simulink model "brakelight_example"  (R2025b)
settings: Solver=FixedStepAuto  StartTime=0.0  StopTime=10.0  RelTol=1e-3
libraries: simulink x3
settings Model: Creator=seanmk  LastModifiedBy=seanmk
settings ConfigComp: DVMaxProcessTime=300.0  DVModelCoverageObjectives=MCDC  DVMaxTestCaseSteps=10000.0  DVTestSuiteOptimization=Auto  DVAbsoluteTolerance=1.0e-5  DVDefectChecker=on  DVDetectOutOfBounds=on  DVMaxViolationSteps=20.0  DVModelReferenceHarness=on  DVHarnessSource=Signal Editor  DVActiveTab=0.0

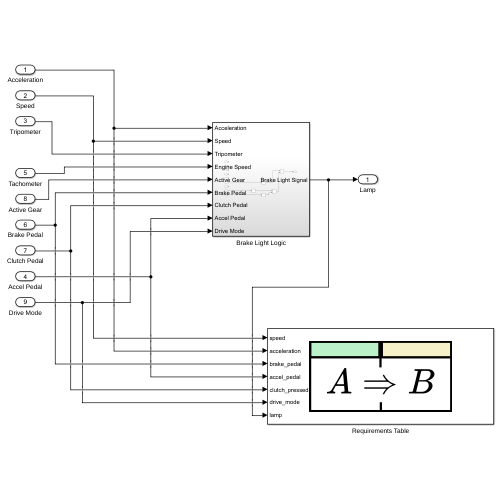
[thumbnail: Simulink's stored preview of the top-level diagram]
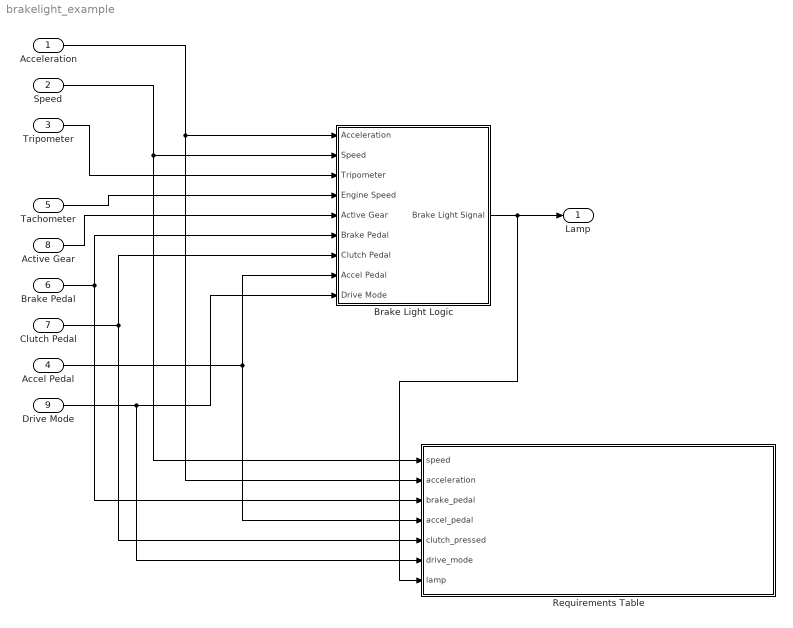
== system brakelight_example ==
  Acceleration : Inport
  Speed : Inport  Port=2
  Tripometer : Inport  Port=3
  Accel Pedal : Inport  Port=4
  Tachometer : Inport  Port=5
  Brake Pedal : Inport  Port=6
  Clutch Pedal : Inport  Port=7
  Active Gear : Inport  Port=8
  Drive Mode : Inport  Port=9
  Brake Light Logic : Subsystem
  Requirements Table : Requirements Table  TreatAsAtomicUnit=on
  Lamp : Outport
  wires:
  Acceleration/1 -> Requirements Table/2(acceleration), Brake Light Logic/1(Acceleration)
  Tripometer/1 -> Brake Light Logic/3(Tripometer)
  Speed/1 -> Brake Light Logic/2(Speed), Requirements Table/1(speed)
  Brake Pedal/1 -> Requirements Table/3(brake_pedal), Brake Light Logic/6(Brake Pedal)
  Clutch Pedal/1 -> Brake Light Logic/7(Clutch Pedal), Requirements Table/5(clutch_pressed)
  Tachometer/1 -> Brake Light Logic/4(Engine Speed)
  Active Gear/1 -> Brake Light Logic/5(Active Gear)
  Accel Pedal/1 -> Requirements Table/4(accel_pedal), Brake Light Logic/8(Accel Pedal)
  Brake Light Logic/1(Brake Light Signal) -> Lamp/1, Requirements Table/7(lamp)
  Drive Mode/1 -> Requirements Table/6(drive_mode), Brake Light Logic/9(Drive Mode)

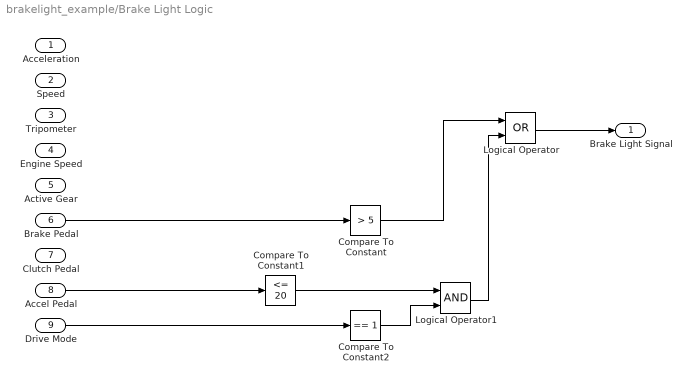
== system brakelight_example/Brake Light Logic ==
  Acceleration : Inport
  Speed : Inport  Port=2
  Tripometer : Inport  Port=3
  Engine Speed : Inport  Port=4
  Active Gear : Inport  Port=5
  Brake Pedal : Inport  Port=6
  Clutch Pedal : Inport  Port=7
  Accel Pedal : Inport  Port=8
  Drive Mode : Inport  Port=9
  Compare To Constant : simulink/Logic and Bit Operations/Compare To Constant  relop=>  const=5  OutDataTypeStr=boolean
  Compare To Constant1 : simulink/Logic and Bit Operations/Compare To Constant  relop=<=  const=20  OutDataTypeStr=boolean
  Compare To Constant2 : simulink/Logic and Bit Operations/Compare To Constant  relop===  const=1  OutDataTypeStr=boolean
  Logical Operator : Logic  Operator=OR  AllPortsSameDT=off  OutDataTypeStr=boolean
  Logical Operator1 : Logic  AllPortsSameDT=off  OutDataTypeStr=boolean
  Brake Light Signal : Outport
  wires:
  Drive Mode/1 -> Compare To Constant2/1
  Brake Pedal/1 -> Compare To Constant/1
  Logical Operator/1 -> Brake Light Signal/1
  Compare To Constant/1 -> Logical Operator/1
  Accel Pedal/1 -> Compare To Constant1/1
  Compare To Constant1/1 -> Logical Operator1/1
  Compare To Constant2/1 -> Logical Operator1/2
  Logical Operator1/1 -> Logical Operator/2

== stateflow chart brakelight_example/Requirements Table ==
  (default) -> (junction 1073742163)
  (junction 1073742163) -> (junction 1073742164) : {
      | % SF_REQ_REV_08
      | }
  (junction 1073742164) -> (junction 1073742166) : {
      | % ExcEvals:
      | % PriEvals:
      | }
  (junction 1073742166) -> (junction 1073742168) : {
      | % HEADER_ASSIGNMENTS
      |
      | }
  (junction 1073742168) -> (junction 1073742170) : {
      | % START_A_4
      | }
  (junction 1073742170) -> (junction 1073742172) : {
      | }
  (junction 1073742172) -> (junction 1073742174)
  (junction 1073742174) -> (junction 1073742176) : {
      | }
  (junction 1073742176) -> (junction 1073742178) : {
      | % END_A_4
      | }
  (junction 1073742178) -> (junction 1073742212) : {
      | % START_R_1
      | }
  (junction 1073742212) -> (junction 1073742214) : {
      | }
  (junction 1073742214) -> (junction 1073742216)
  (junction 1073742216) -> (junction 1073742218) [order 1] : [(brake_pedal > 5)]
  (junction 1073742216) -> (junction 1073742224) [order 2]
  (junction 1073742218) -> (junction 1073742220) : {
      | reqtable_postcondition((lamp == true), 'R:1');
      |
      |
      | }
  (junction 1073742220) -> (junction 1073742222) : {
      | }
  (junction 1073742222) -> (junction 1073742224)
  (junction 1073742224) -> (junction 1073742226)
  (junction 1073742226) -> (junction 1073742228) : {
      | % END_R_1
      | }
  (junction 1073742228) -> (junction 1073742233) : {
      | % START_R_7
      | }
  (junction 1073742233) -> (junction 1073742235) : {
      | }
  (junction 1073742235) -> (junction 1073742237)
  (junction 1073742237) -> (junction 1073742239) [order 1] : [(drive_mode == 1 && accel_pedal <= 20)]
  (junction 1073742237) -> (junction 1073742245) [order 2]
  (junction 1073742239) -> (junction 1073742241) : {
      | reqtable_postcondition((lamp == true), 'R:2');
      |
      |
      | }
  (junction 1073742241) -> (junction 1073742243) : {
      | }
  (junction 1073742243) -> (junction 1073742245)
  (junction 1073742245) -> (junction 1073742247)
  (junction 1073742247) -> (junction 1073742249) : {
      | % END_R_7
      | }
  (junction 1073742249) -> (junction 1073742254) : {
      | % START_R_10
      | }
  (junction 1073742254) -> (junction 1073742256) : {
      | }
  (junction 1073742256) -> (junction 1073742258)
  (junction 1073742258) -> (junction 1073742260) [order 1] : [(drive_mode ~= 1 && brake_pedal <= 5)]
  (junction 1073742258) -> (junction 1073742266) [order 2]
  (junction 1073742260) -> (junction 1073742262) : {
      | reqtable_postcondition((lamp == false), 'R:3');
      |
      |
      | }
  (junction 1073742262) -> (junction 1073742264) : {
      | }
  (junction 1073742264) -> (junction 1073742266)
  (junction 1073742266) -> (junction 1073742268)
  (junction 1073742268) -> (junction 1073742270) : {
      | % END_R_10
      | }
  (junction 1073742270) -> (junction 1073742287) : {
      | % START_R_13
      | }
  (junction 1073742287) -> (junction 1073742289) : {
      | }
  (junction 1073742289) -> (junction 1073742291)
  (junction 1073742291) -> (junction 1073742293) [order 1] : [(drive_mode == 1 && brake_pedal < 5 && accel_pedal > 20)]
  (junction 1073742291) -> (junction 1073742299) [order 2]
  (junction 1073742293) -> (junction 1073742295) : {
      | reqtable_postcondition((lamp == false), 'R:4');
      |
      |
      | }
  (junction 1073742295) -> (junction 1073742297) : {
      | }
  (junction 1073742297) -> (junction 1073742299)
  (junction 1073742299) -> (junction 1073742301)
  (junction 1073742301) -> (junction 1073742303) : {
      | % END_R_13
      | }
  data: speed input; acceleration input; brake_pedal input; accel_pedal input; clutch_pressed input; drive_mode input; lamp input
